simulink model "MIMO_BPSK_Alamouti"  (R2026a)
settings: Solver=FixedStepDiscrete  StopTime=1/PayloadBitRate*560*300  FixedStep=1/PayloadBitRate*560
PreLoadFcn:
  | PayloadBitRate = 250e3/4;
  | EbNo = 15;
  | modHeader = pskmod([1 1 1 1 1 0 0 1 1 0 1 0 1].', 2, 0);
model workspace: external: MAT-File modelspace.mat (data not in the file)
undefined symbols (not defined in the file or in its folder): doppler, gcbh, rcfiltgaincompat
libraries: commchan3 x3, commrflib2 x3, commrfcorlib x2, commmimo x2, commdigbbndpm3 x2, commsync2 x2, commfilt2 x2
settings Model: LastModifiedBy=hcha7553
settings DataIOCC: SignalLoggingSaveFormat=ModelDataLogs
settings DebuggingCC: UnderspecifiedInitializationDetection=Classic
settings HardwareCC: ProdHWDeviceType=32-bit Generic
settings GRTTargetCC: CombineOutputUpdateFcns=off  GRTInterface=on

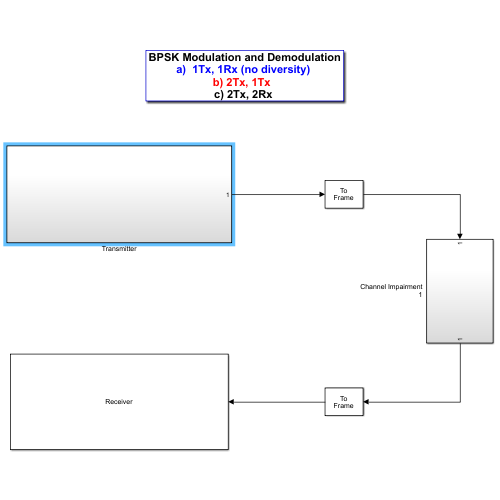
[thumbnail: Simulink's stored preview of the top-level diagram]
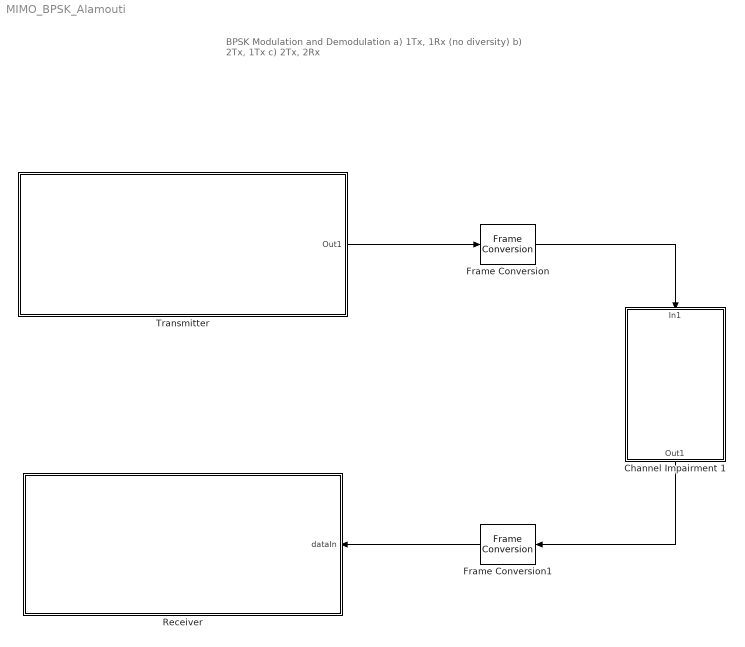
== system MIMO_BPSK_Alamouti ==
  note: BPSK Modulation and Demodulation
      | a) 1Tx, 1Rx (no diversity)
      | b) 2Tx, 1Tx
      | c) 2Tx, 2Rx
  Channel Impairment 1 : Subsystem
  Frame Conversion : FrameConversion
  Frame Conversion1 : FrameConversion
  Receiver : Subsystem
      mask Display: disp('Receiver')
  Transmitter : Subsystem
  wires:
  Transmitter/1(Out1) -> Frame Conversion/1
  Frame Conversion1/1 -> Receiver/1(dataIn)
  Frame Conversion/1 -> Channel Impairment 1/1(In1)
  Channel Impairment 1/1(Out1) -> Frame Conversion1/1

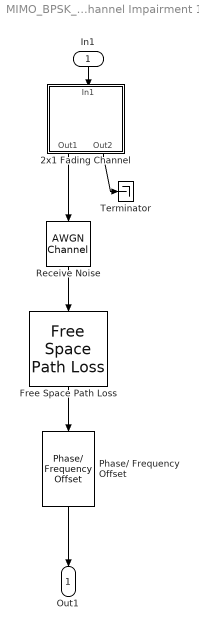
== system MIMO_BPSK_Alamouti/Channel Impairment 1 ==
  In1 : Inport
  2x1 Fading Channel : Subsystem
      mask Display: disp('2 x 1\nFading\nChannel');
  Free Space Path Loss : commrflib2/Free Space Path Loss  mode=Decibels  dB=25  d=0.100  fc=1920
  Phase/ Frequency Offset : commrflib2/Phase// Frequency Offset  phaseOffset=47  freqPort=off  freqOffset=5000
  Receive Noise : commchan3/AWGN Channel  LegacyMode=on  NoiseMethod="Signal to noise ratio  (SNR)"  noiseMode="Signal to noise ratio  (Es/No)"  EbNo=EbNo-10*log10(4)  EsNo=EbNo  SNR=EbNo  BitsPerSymbol=4  SignalPower=2  SamplesPerSymbol=1  SymbolPeriod=1/(PayloadBitRate)*560/2324  VarianceSource=Parameter  Variance=1  RandomStream=Global stream  Seed=188  SimulateUsing=Code generation
  Terminator : Terminator
  Out1 : Outport  VectorParamsAs1DForOutWhenUnconnected=off
  wires:
  In1/1 -> 2x1 Fading Channel/1(In1)
  Receive Noise/1 -> Free Space Path Loss/1
  2x1 Fading Channel/2(Out2) -> Terminator/1
  Phase/ Frequency Offset/1 -> Out1/1
  Free Space Path Loss/1 -> Phase/ Frequency Offset/1
  2x1 Fading Channel/1(Out1) -> Receive Noise/1

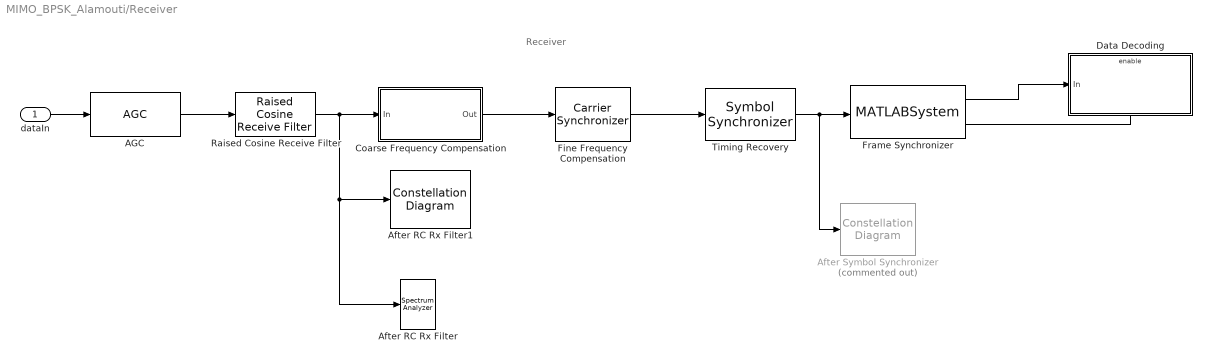
== system MIMO_BPSK_Alamouti/Receiver ==
  note: Receiver
  dataIn : Inport
  AGC : commrfcorlib/AGC  LegacyMode=off  DetectorMethod=Rectifier  LoopMethod=Linear  UpdatePeriod=100  StepSize=0.1  AdaptationStepSize=0.01  DesiredOutputPower=1/sqrt(4)/2  AveragingLength=2324  MaximumGain=30  MaxPowerGain=50  GainOutputPort=off  InputPowerOutputPort=off  SimulateUsing=Code generation
  After RC Rx Filter : SpectrumAnalyzer  WindowPosition=[1028.000000,469.000000,800.000000,500.000000,]  ScopeFrameLocation=window  Method=Welch  SampleRate=129687.5  RBWSource=Property  RBW=75  FFTLength=128  Span=100000  StartFrequency=-50000  StopFrequency=50000  AveragingMethod=Running  SpectralAverages=2  SpectrumUnits=dBW  Title=After Raised Cosine Rx Filter  YLabel=Power Spectrum  YLimits=[-116.98239536,-2.24819024]  ShowGrid=off  AllowFFTLengthLessThanSamplesPerUpdate=on  DefaultConfigurationName=spbscopes.SpectrumAnalyzerBlockCfg  IsFrequencyInputMode=0  FrequencyVectorPort=0  FrequencyVectorFromPort=0  FrequencyInputRBWPort=0  FrequencyInputRBWFromPort=0
  After RC Rx Filter1 : ConstellationDiagram  Tag=ScatterPlot  WindowPosition=[1057.000000,180.000000,401.000000,517.000000,]  ScopeFrameLocation=window  SamplesPerSymbol=2  SymbolsToDisplaySource=Property  SymbolsToDisplay=1000  ReferenceConstellation=BPSK  Title=After Raised Cosine Rx Filter  XLimits=[-1.25 1.25]  YLimits=[-1.25 1.25]  AxesLimits=[-1.25 1.25]  DefaultConfigurationName=comm.scopes.ConstellationDiagramBlockCfg
  After Symbol Synchronizer : ConstellationDiagram  Tag=ScatterPlot  Commented=on  WindowPosition=[1436.000000,665.000000,403.000000,337.000000,]  Visible=on  ScopeFrameLocation=window  SamplesPerSymbol=2  SymbolsToDisplaySource=Property  SymbolsToDisplay=1000  ReferenceConstellation=BPSK  Title=After Symbol Synchronizer  XLimits=[-1.25 1.25]  YLimits=[-1.25 1.25]  AxesLimits=[-1.25 1.25]  DefaultConfigurationName=comm.scopes.ConstellationDiagramBlockCfg
  Coarse Frequency Compensation : Subsystem
      mask Display: disp('Coarse Frequency\nCompensation');
  Data Decoding : Subsystem
      mask Display: disp('Data Decoding');
  Fine Frequency Compensation : commsync2/Carrier Synchronizer  Modulation=BPSK  ModulationPhaseOffset=Custom  CustomPhaseOffset=0  SamplesPerSymbol=2  DampingFactor=1  NormalizedLoopBandwidth=0.01  EstimatedPhaseErrorOutputPort=off  SimulateUsing=Code generation
  Frame Synchronizer : MATLABSystem  System=FrameFormation  OutputFrameLength=581  PerformSynchronization=on  InternalBufferLength=300  FrameHeader=modHeader  SimulateUsing=Interpreted execution
      mask Type: FrameFormation
  Raised Cosine Receive Filter : commfilt2/Raised Cosine Receive Filter  filtType=Square root  R=0.5  filtSpan=10  N=4  downFactor=2  downOffset=0  filterGain=rcfiltgaincompat(gcbh)  InputProcessing=Columns as channels (frame based)  RateOptions=Enforce single-rate processing  framing=Enforce single-rate processing  checkCoeff=off  variableName=rcRxFilt1  currentFiltSpan=10  D=(10)/2  inputOffset=0  sampMode=Mute  saveAsFlag=0  rateMode=Downsampling  checkGain=Normalized  launchFVT=off  roundingMode=Floor  overflowMode=off  coeffDataTypeStr=Inherit: Same word length as input  coeffMin=[]  coeffMax=[]  coeffLastDataTypeStr=Inherit: Same word length as input  accumDataTypeStr=Inherit: Same as product output  accumLastDataTypeStr=Inherit: Same as product output  outputDataTypeStr=Inherit: Same as accumulator  outputMin=[]  outputMax=[]  outputLastDataTypeStr=Inherit: Same as accumulator
  Timing Recovery : commsync2/Symbol Synchronizer  Modulation=PAM/PSK/QAM  TimingErrorDetector=Early-Late (non-data-aided)  SamplesPerSymbol=2  DampingFactor=1  NormalizedLoopBandwidth=0.01  DetectorGain=5.4  TimingErrorOutputPort=off  SimulateUsing=Code generation
  wires:
  Frame Synchronizer/1 -> Data Decoding/1(In)
  Frame Synchronizer/2 -> Data Decoding/Enable
  Raised Cosine Receive Filter/1 -> Coarse Frequency Compensation/1(In), After RC Rx Filter1/1, After RC Rx Filter/1
  Coarse Frequency Compensation/1(Out) -> Fine Frequency Compensation/1
  Fine Frequency Compensation/1 -> Timing Recovery/1
  dataIn/1 -> AGC/1
  AGC/1 -> Raised Cosine Receive Filter/1
  Timing Recovery/1 -> Frame Synchronizer/1, After Symbol Synchronizer/1

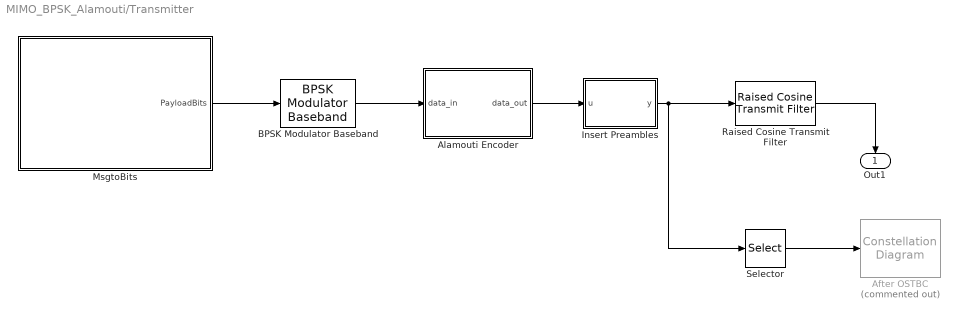
== system MIMO_BPSK_Alamouti/Transmitter ==
  After OSTBC : ConstellationDiagram  Tag=ScatterPlot  Commented=on  WindowPosition=[404.000000,311.000000,600.000000,600.000000,]  Visible=on  ScopeFrameLocation=window  SamplesPerSymbol=2  SymbolsToDisplaySource=Property  SymbolsToDisplay=1000  ReferenceConstellation=BPSK  Title=After Raised Cosine Rx Filter  XLimits=[-1.25 1.25]  YLimits=[-1.25 1.25]  AxesLimits=[-1.25 1.25]  DefaultConfigurationName=comm.scopes.ConstellationDiagramBlockCfg
  Alamouti Encoder : Subsystem  mask(Constant){Select_1=2}
      mask prompts: Select_1 "Encoder Selection"
      mask help:
      | Encoder Selection Parameter:
      | 1 Simulink Block
      | 2 User Defined Function
      mask init:
      | Select=1
  BPSK Modulator Baseband : commdigbbndpm3/BPSK Modulator Baseband  Ph=0  outDtype=double  outWordLen=16  outUDDataType=sfix(16)  outFracLenMode=Best precision  outFracLen=15  outDataTypeStr=double  outLastDataTypeStr=double
  Insert Preambles : MATLAB Function  TreatAsAtomicUnit=on
  MsgtoBits : MATLAB Function  TreatAsAtomicUnit=on
  Raised Cosine Transmit Filter : commfilt2/Raised Cosine Transmit Filter  filtType=Square root  R=0.5  filtSpan=10  N=4  filterGain=rcfiltgaincompat(gcbh)  InputProcessing=Columns as channels (frame based)  RateOptions=Enforce single-rate processing  framing=Mute  checkCoeff=off  variableName=rcTxFilt  checkGain=Normalized  sampMode=Mute  saveAsFlag=0  currentFiltSpan=10  D=(10)/2  launchFVT=off  roundingMode=Floor  overflowMode=off  coeffDataTypeStr=Inherit: Same word length as input  coeffMin=[]  coeffMax=[]  coeffLastDataTypeStr=Inherit: Same word length as input  outputDataTypeStr=Inherit: Same as accumulator  outputMin=[]  outputMax=[]  outputLastDataTypeStr=Inherit: Same as accumulator
  Selector : Selector  NumberOfDimensions=2  InputPortWidth=3  IndexOptions=Select all,Index vector (dialog)  Indices=[1 3],1  OutputSizes=1,1
  Out1 : Outport  VectorParamsAs1DForOutWhenUnconnected=off
  wires:
  Insert Preambles/1(y) -> Raised Cosine Transmit Filter/1, Selector/1
  BPSK Modulator Baseband/1 -> Alamouti Encoder/1(data_in)
  MsgtoBits/1(PayloadBits) -> BPSK Modulator Baseband/1
  Alamouti Encoder/1(data_out) -> Insert Preambles/1(u)
  Raised Cosine Transmit Filter/1 -> Out1/1
  Selector/1 -> After OSTBC/1

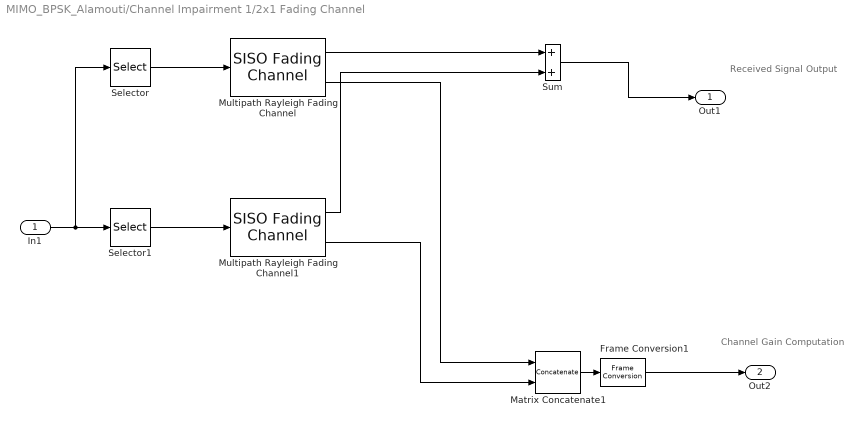
== system MIMO_BPSK_Alamouti/Channel Impairment 1/2x1 Fading Channel ==
  note: Channel Gain Computation
  note: Received Signal Output
  In1 : Inport
  Frame Conversion1 : FrameConversion  OutFrame=Sample-based
  Matrix Concatenate1 : Concatenate  Mode=Multidimensional array  ConcatenateDimension=2
  Multipath Rayleigh Fading Channel : commchan3/SISO Fading Channel  InheritSampleRate=on  SampleRate=1  PathDelays=0  AveragePathGains=0  NormalizePathGains=on  FadingDistribution=Rayleigh  KFactor=3  DirectPathDopplerShift=0  DirectPathInitialPhase=0  MaximumDopplerShift=1  DopplerSpectrum=doppler('Jakes')  RandomStream=mt19937ar with seed  Seed=12345  PathGainsOutputPort=on  ChannelFilterDelayOutputPort=off  SimulateUsing=Interpreted execution  Visualization=Off  PathsForDopplerDisplay=1  SamplesToDisplay=25%
  Multipath Rayleigh Fading Channel1 : commchan3/SISO Fading Channel  InheritSampleRate=on  SampleRate=1  PathDelays=0  AveragePathGains=0  NormalizePathGains=on  FadingDistribution=Rayleigh  KFactor=3  DirectPathDopplerShift=0  DirectPathInitialPhase=0  MaximumDopplerShift=1  DopplerSpectrum=doppler('Jakes')  RandomStream=mt19937ar with seed  Seed=24680  PathGainsOutputPort=on  ChannelFilterDelayOutputPort=off  SimulateUsing=Interpreted execution  Visualization=Off  PathsForDopplerDisplay=1  SamplesToDisplay=25%
  Selector : Selector  NumberOfDimensions=2  InputPortWidth=3  IndexOptions=Select all,Index vector (dialog)  Indices=-1,1  OutputSizes=1
  Selector1 : Selector  NumberOfDimensions=2  InputPortWidth=3  IndexOptions=Select all,Index vector (dialog)  Indices=-1,2  OutputSizes=1
  Sum : Sum
  Out1 : Outport  VectorParamsAs1DForOutWhenUnconnected=off
  Out2 : Outport  Port=2  VectorParamsAs1DForOutWhenUnconnected=off
  wires:
  Frame Conversion1/1 -> Out2/1
  Matrix Concatenate1/1 -> Frame Conversion1/1
  Sum/1 -> Out1/1
  Selector/1 -> Multipath Rayleigh Fading Channel/1
  Selector1/1 -> Multipath Rayleigh Fading Channel1/1
  Multipath Rayleigh Fading Channel/2 -> Matrix Concatenate1/1
  Multipath Rayleigh Fading Channel1/2 -> Matrix Concatenate1/2
  Multipath Rayleigh Fading Channel/1 -> Sum/1
  Multipath Rayleigh Fading Channel1/1 -> Sum/2
  In1/1 -> Selector/1, Selector1/1

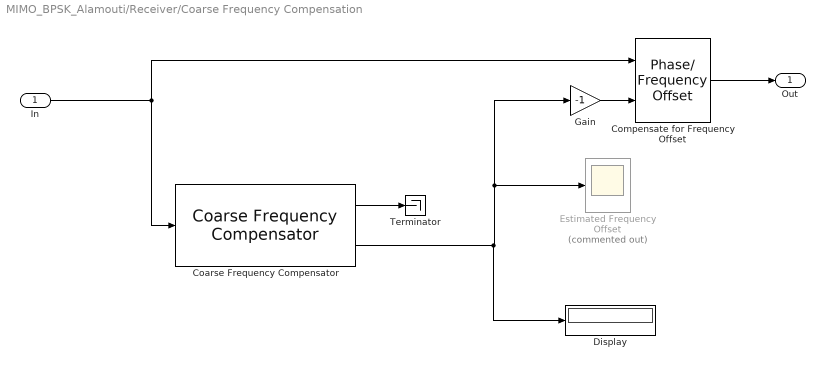
== system MIMO_BPSK_Alamouti/Receiver/Coarse Frequency Compensation ==
  In : Inport
  Coarse Frequency Compensator : commrfcorlib/Coarse Frequency Compensator  Modulation=BPSK  Algorithm=FFT-based  FrequencyResolution=50  MaximumFrequencyOffset=5e3  SamplesPerSymbol=4  EstimatedFreqOffsetPort=on  SimulateUsing=Code generation
  Compensate for Frequency Offset : commrflib2/Phase// Frequency Offset  phaseOffset=0  freqPort=on  freqOffset=100
  Display : Display
  Estimated Frequency Offset : Scope  Commented=on
      settings: TimeSpan=0.1  TimeUnits=Metric (based on Time Span)  ActiveDisplayYMinimum=4004.88  ActiveDisplayYMaximum=6004.88  YLabel=Estimated Frequency Offset (Hz)  DataLoggingVariableName=ScopeDataEFO
  Gain : Gain  Gain=-1
  Terminator : Terminator
  Out : Outport  VectorParamsAs1DForOutWhenUnconnected=off
  wires:
  In/1 -> Coarse Frequency Compensator/1, Compensate for Frequency Offset/1
  Compensate for Frequency Offset/1 -> Out/1
  Gain/1 -> Compensate for Frequency Offset/2
  Coarse Frequency Compensator/1 -> Terminator/1
  Coarse Frequency Compensator/2 -> Display/1, Estimated Frequency Offset/1, Gain/1

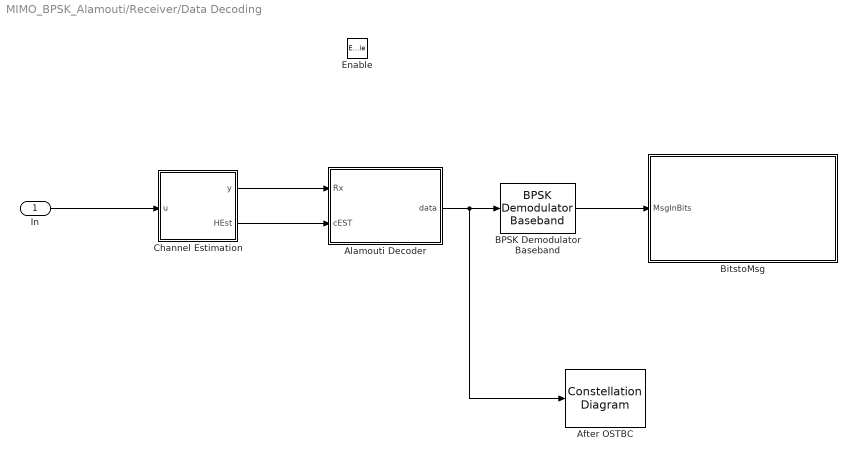
== system MIMO_BPSK_Alamouti/Receiver/Data Decoding ==
  In : Inport
  Enable : EnablePort
  After OSTBC : ConstellationDiagram  Tag=ScatterPlot  WindowPosition=[1488.000000,133.000000,285.000000,338.000000,]  ScopeFrameLocation=window  SamplesPerSymbol=2  SymbolsToDisplaySource=Property  SymbolsToDisplay=1000  ReferenceConstellation=BPSK  Title=After Space time coding  XLimits=[-2.876 2.8997]  YLimits=[-2.876 2.8997]  AxesLimits=[-2.876 2.8997]  ShowLegend=on  DefaultConfigurationName=comm.scopes.ConstellationDiagramBlockCfg
  Alamouti Decoder : Subsystem  mask(Constant){Select_2=2}
      mask prompts: Select_2 "Decoder Selection"
      mask help:
      | Decoder Selection Parameter
      | 1 Simulink Block
      | 2 User Defined Function
  BPSK Demodulator Baseband : commdigbbndpm3/BPSK Demodulator Baseband  DecType=Hard decision  VarSource=Dialog  Variance=1  Ph=0  outDtype=double  derotateFactorWordLen=16  derotateFactorDataTypeStr=Inherit: Same word length as input  derotateFactorLastDataTypeStr=Inherit: Same word length as input
  BitstoMsg : MATLAB Function  TreatAsAtomicUnit=on
  Channel Estimation : MATLAB Function  TreatAsAtomicUnit=on
  wires:
  In/1 -> Channel Estimation/1(u)
  Alamouti Decoder/1(data) -> After OSTBC/1, BPSK Demodulator Baseband/1
  Channel Estimation/1(y) -> Alamouti Decoder/1(Rx)
  Channel Estimation/2(HEst) -> Alamouti Decoder/2(cEST)
  BPSK Demodulator Baseband/1 -> BitstoMsg/1(MsgInBits)

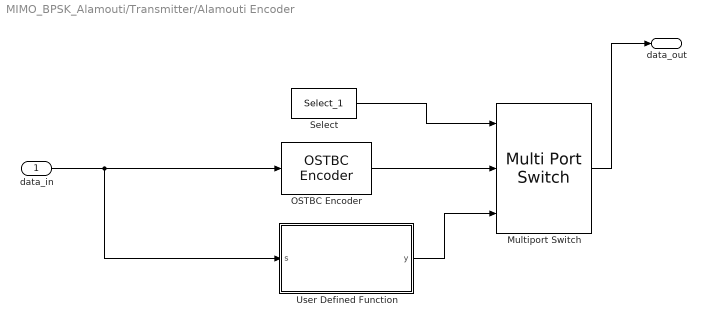
== system MIMO_BPSK_Alamouti/Transmitter/Alamouti Encoder ==
  data_in : Inport
  Multiport Switch : MultiPortSwitch  Inputs=2  SaturateOnIntegerOverflow=off  InputSameDT=off
  OSTBC Encoder : commmimo/OSTBC Encoder  numTx=2  rate=3/4  overflowMode=Wrap  OvFlMode=off  OvFlModeLastStrValue=off
  Select : Constant  Value=Select_1  VectorParams1D=off  OutMin=1  OutMax=5  OutDataTypeStr=Inherit: Inherit via back propagation
  "User Defined Function " : MATLAB Function  TreatAsAtomicUnit=on
  data_out : Outport  VectorParamsAs1DForOutWhenUnconnected=off
  wires:
  data_in/1 -> "User Defined Function "/1(s), OSTBC Encoder/1
  Select/1 -> Multiport Switch/1
  OSTBC Encoder/1 -> Multiport Switch/2
  "User Defined Function "/1(y) -> Multiport Switch/3
  Multiport Switch/1 -> data_out/1

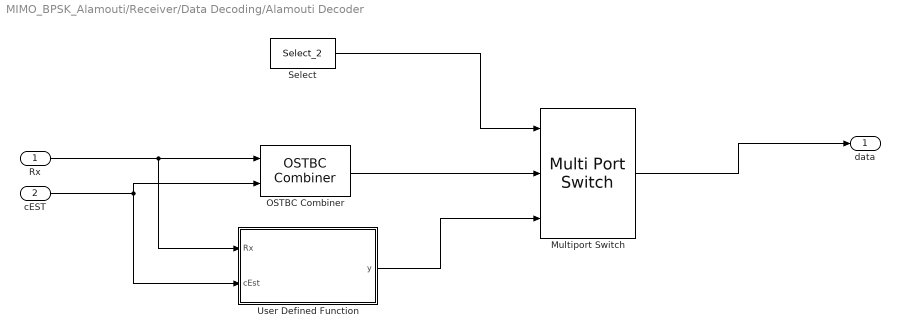
== system MIMO_BPSK_Alamouti/Receiver/Data Decoding/Alamouti Decoder ==
  Rx : Inport
  cEST : Inport  Port=2
  Multiport Switch : MultiPortSwitch  Inputs=2  SaturateOnIntegerOverflow=off  InputSameDT=off
  OSTBC Combiner : commmimo/OSTBC Combiner  numTx=2  rate=3/4  numRx=1  roundingMode=Floor  overflowMode=Wrap  OvFlMode=off  OvFlModeLastStrValue=off  crossProductWordLen=32  crossProductFracLen=16  crossSumWordLen=32  crossSumFracLen=16  egyProductWordLen=32  egyProductFracLen=16  egySumWordLen=32  egySumFracLen=16  divisionWordLen=32  divisionFracLen=16  divisionDataTypeStr=Inherit: Same as accumulator  divisionLastDataTypeStr=Inherit: Same as accumulator
  Select : Constant  Value=Select_2  VectorParams1D=off  OutMin=1  OutMax=5  OutDataTypeStr=Inherit: Inherit via back propagation
  "User Defined Function " : MATLAB Function  TreatAsAtomicUnit=on
  data : Outport  VectorParamsAs1DForOutWhenUnconnected=off
  wires:
  Select/1 -> Multiport Switch/1
  Rx/1 -> OSTBC Combiner/1, "User Defined Function "/1(Rx)
  cEST/1 -> OSTBC Combiner/2, "User Defined Function "/2(cEst)
  OSTBC Combiner/1 -> Multiport Switch/2
  "User Defined Function "/1(y) -> Multiport Switch/3
  Multiport Switch/1 -> data/1

== matlab function MIMO_BPSK_Alamouti/Receiver/Data Decoding/Channel Estimation ==
  data: u input; y output size=[560, 1]; HEst output
function [y, HEst] = fcn(u)
%incomplete code
HEst = complex(zeros(560, 2));
y=u(22:581);

== matlab function MIMO_BPSK_Alamouti/Transmitter/Insert Preambles ==
  data: u input; y output
function y = fcn(u)
%incomplete code
modBarkerCode=zeros(13,1);  
pilots=zeros(8,2);

% preamble construction for MIMO 2 RF Transmitter
y = [[modBarkerCode ,modBarkerCode];pilots; u];

== matlab function MIMO_BPSK_Alamouti/Transmitter/Alamouti Encoder/User Defined Function  ==
  data: s input; y output size=[560, 2]
function y = Alamouti_encoder(s)
%incomplete code
y=complex(zeros(560,2));

== matlab function MIMO_BPSK_Alamouti/Transmitter/MsgtoBits ==
  data: PayloadBits output double size=[560, 1]
function PayloadBits   = MsgtoBits
%This function converts a message to payloadBits with padding 

%% Configuration paramters
%System Paramters
   NumBitsPerCharacter  = 7;
   
%% Alogrithm 
%Payload message
    PayloadMessage = 'Welcome to the school of electrical and information engineering, Uni. of Sydney!';
    %PayloadMessage = zeros(80,1) +127;
    
%Convert message to bits
    coder.extrinsic('dec2bin');
    msgInBits = coder.const(double(dec2bin(PayloadMessage, NumBitsPerCharacter).'));
    PayloadBits = msgInBits(:) - 48;

== matlab function MIMO_BPSK_Alamouti/Receiver/Data Decoding/Alamouti Decoder/User Defined Function  ==
  data: Rx input; y output size=[560, 1]; cEst input
function y = Alamouti_decoder(Rx, cEst)
%incomplete code
y=complex(zeros(560,1));

== matlab function MIMO_BPSK_Alamouti/Receiver/Data Decoding/BitstoMsg ==
  data: MsgInBits input; NumFrameDetected data_store_memory; SystemBER data_store_memory
function BitstoMsg(MsgInBits)

% Configuration paramters
PayloadMessage = 'Welcome to the school of electrical and information engineering, Uni. of Sydney!';
NumBitsPerCharacter  = 7;
global NumFrameDetected;    %count the number of frame correctly received
global SystemBER;
coder.extrinsic('dec2bin','fprintf','num2str');
%% Alorithm

NumFrameDetected=NumFrameDetected+1;     
if NumFrameDetected <= 200 && NumFrameDetected>1 %only display first 200 frame, avoid channel sample cut
    % transmitted message

    txMsgInBits    = coder.const(double(dec2bin(PayloadMessage, NumBitsPerCharacter).'));
    txMsgInBits    = txMsgInBits(:) - 48;
    bitMsgLen      = length(txMsgInBits);

    % received message
    %remove padding
    rxMsgInBits = MsgInBits(1:bitMsgLen,:);
    % disp(rxMsgInBits);
    decMsgInBits = reshape(rxMsgInBits(1:bitMsgLen),[7, bitMsgLen/7])';
    %decMsgInBits = reshape(rxMsgInBits(1:bitMsgLen),[bitMsgLen/7, 7]);
    disp('Received Message:');
    disp(char(bin2dec(num2str(decMsgInBits)))');

    %% BER
    % BER calculation
    numBitErr = sum(txMsgInBits(:) ~= rxMsgInBits(:));
    BER = numBitErr/(bitMsgLen);
    
    SystemBER = (SystemBER*(NumFrameDetected-1) + BER)/NumFrameDetected;%accumulated BER
    fprintf('Error Stats:\nTotal number of Frame detected = %d.  The System average BER = %f\n\n', ...
             NumFrameDetected, SystemBER);
 end
